simulink model "sm_excv_track1"  (R2026b)
settings: Solver=ode23t  StopTime=14  FixedStep=2e-4  AbsTol=1e-3
StartFcn:
  | tic
StopFcn:
  | Elapsed_Sim_Time = toc;
  | disp(['Elapsed Sim Time = ' num2str(Elapsed_Sim_Time)]);
undefined symbols (not defined in the file): Excv, X, Y, Z
libraries: sm_trackV_lib_terrain_contact x4, sm_lib x3, fl_lib x2, sm_excv_chassis_lib x2, nesl_utility x2, sm_trackV_lib_chain_underc_elem x1, sm_trackV_lib_chain_lower_frame_s46i1u2l7 x1, simulink x1
CloseFcn:
  | try,close(h1_sm_excv_track_single_terrain),end
  | clear h1_sm_excv_track_single_terrain
  | try,close(h2_sm_excv_track_single_terrain),end
  | clear h2_sm_excv_track_single_terrain
  | try,close(h3_sm_excv_track_single_terrain),end
  | clear h3_sm_excv_track_single_terrain
  | try,close(h4_sm_excv_track_single_terrain),end
  | clear h4_sm_excv_track_single_terrain
  | 
  | 
  | %clear simlog_sm_excv_track_single_road_plate
  | %clear logsout_sm_excv_track_single_road_plate
settings Model: Creator=evo  LastModifiedBy=smiller
settings SolverCC: AutoScaleAbsTol=off
settings DataIOCC: DSMLogging=off  ReturnWorkspaceOutputs=off  SaveOutput=off  SaveTime=off  SignalLoggingName=logsout_sm_excv_track1
settings DebuggingCC: SymbolicDimsDataTypeCodeGenerationDiagnostic=none
settings SFSimCC: CustomCodeUndefinedFunction=UseInterfaceOnly
settings RTWCC: DLArmComputeVersion=19.05
settings SimscapeCC: SimscapeLogLimitData=off  SimscapeLogName=simlog_sm_excv_track1  SimscapeLogSimulationStatistics=on  SimscapeLogType=all  SimscapeUseEnergyAccounting=off
settings DiagnosticsConfigSet: SimMechanicsConflictingReferenceFrames=none
settings ExplorerConfigSet: InternalSimMechanicsExplorerSettings="<ExplorerConfiguration><canonicalview>default</canonicalview><AnimationSetting><BasePlaybackSpeed>1.0</BasePlaybackSpeed><PlaybackSpeedFactor>0.25</PlaybackSpeedFactor></AnimationSetting><TilePanel><TileInfo><Tiles Columns=\"2\" Count=\"3\" Rows=\"2\"><Column Weight=\"0.5\"/><Column Weight=\"0.5\"/><Row Weight=\"0.5\"/><Row Weight=\"0.5\"/><Tile Height=\"1\" Width=\"2\" X=\"0\" Y=\"0\"/><Tile Height=\"1\" Width=\"1\" X=\"0\" Y=\"1\"/><Tile Height=\"1\" Width=\"1\" X=\"1\" Y=\"1\"/></Tiles></TileInfo><SceneInfo><SceneViewer><BGColor><R>1</R><G>1</G><B>1</B></BGColor><Camera><DoPerspective>on</DoPerspective><Position><X>4.57499999999987139</X><Y>-0.500000000001179279</Y><Z>0.554946553288407585</Z></Position><Center><X>4.15238173825940571</X><Y>0.406307787035579571</Y><Z>0.554946553288434119</Z></Center><Up><X>0</X><Y>0</Y><Z>1</Z></Up><ViewLimDist>1</ViewLimDist><YLim>0.466307658154998583</YLim><XLim>0.887968838401539839</XLim></Camera></SceneViewer><SceneViewer><BGColor><R>1</R><G>1</G><B>1</B></BGColor><Camera><DoPerspective>off</DoPerspective><Position><X>10.0004286080142499</X><Y>-63.1345143988139412</Y><Z>2.01677578846033079</Z></Position><Center><X>10.0000005340652702</X><Y>2.24533280857031059e-10</Y><Z>0.750000011139050793</Z></Center><Up><X>0.000675779963889239091</X><Y>0.0200606731361765434</Y><Z>0.999798536063523424</Z></Up><ViewLimDist>1</ViewLimDist><YLim>11.3757180156657967</YLim><XLim>10.6496083550913845</XLim></Camera></SceneViewer><SceneViewer><BGColor><R>1</R><G>1</G><B>1</B></BGColor><Camera><DoPerspective>on</DoPerspective><Position><X>1.68499999999974204</X><Y>-1.00000000000043432</Y><Z>0.55494655328839293</Z></Position><Center><X>1.68500000000000005</X><Y>-4.34319247233361239e-13</Y><Z>0.55494655328842224</Z></Center><Up><X>0</X><Y>0</Y><Z>1</Z></Up><ViewLimDist>1</ViewLimDist><YLim>0.466307658154998583</YLim><XLim>0.436543339549360365</XLim></Camera></SceneViewer></SceneInfo></TilePanel><MechEditorPanel><Cameras><Camera><Id>Camera1</Id><Value><Name>Track_CtrRear_AimFront</Name><NativeCamera><PositionTrackingFeature>Chassis.Camera_Frames.CamF_CtrRear_AimLF.R</PositionTrackingFeature><CenterTrackingFeature>Config.World_Frame.W</CenterTrackingFeature><UpVectorTrackingFeature>Config.World_Frame.W</UpVectorTrackingFeature><CenterTrackingOrigin>off</CenterTrackingOrigin><CenterTrackingDirection>+X</CenterTrackingDirection><UpVectorTrackingDirection>+Z</UpVectorTrackingDirection></NativeCamera></Value></Camera><Camera><Id>Camera2</Id><Value><Name>Track_Left_AimRight</Name><NativeCamera><PositionTrackingFeature>Chassis.Camera_Frames.CamF_Left_AimRight.R</PositionTrackingFeature><CenterTrackingFeature>Chassis.Camera_Frames.CamF_Left_AimRight.R</CenterTrackingFeature><UpVectorTrackingFeature>Config.World_Frame.W</UpVectorTrackingFeature><CenterTrackingOrigin>off</CenterTrackingOrigin><CenterTrackingDirection>+X</CenterTrackingDirection><UpVectorTrackingDirection>+Z</UpVectorTrackingDirection></NativeCamera></Value></Camera><Camera><Id>Camera3</Id><Value><Name>Track_Front_AimLR</Name><NativeCamera><PositionTrackingFeature>Chassis.Camera_Frames.CamF_Front_AimLR.R</PositionTrackingFeature><CenterTrackingFeature>Chassis.Camera_Frames.Transform_Aim_LR.F</CenterTrackingFeature><UpVectorTrackingFeature>Config.World_Frame.W</UpVectorTrackingFeature><CenterTrackingOrigin>off</CenterTrackingOrigin><CenterTrackingDirection>+X</CenterTrackingDirection><UpVectorTrackingDirection>+Z</UpVectorTrackingDirection></NativeCamera></Value></Camera><Camera><Id>Camera4</Id><Value><Name>Track_Right_AimLeftTL</Name><NativeCamera><PositionTrackingFeature>Chassis.Camera_Frames.CamF_Right_AimLeftTL.R</PositionTrackingFeature><CenterTrackingFeature>Chassis.Camera_Frames.CamF_Right_AimLeftTL.R</CenterTrackingFeature><UpVectorTrackingFeature>Config.World_Frame.W</UpVectorTrackingFeature><CenterTrackingOrigin>off</CenterTrackingOrigin><CenterTrackingDirection>+X</CenterTrackingDirection><UpVectorTrackingDirection>+Z</UpVectorTrackingDirection></NativeCamera></Value></Camera><Camera><Id>Camera5</Id><Value><Name>Track_Right_AimLeftTR</Name><NativeCamera><PositionTrackingFeature>Chassis.Camera_Frames.CamF_Right_AimLeftTR.R</PositionTrackingFeature><CenterTrackingFeature>Chassis.Camera_Frames.CamF_Right_AimLeftTR.R</CenterTrackingFeature><UpVectorTrackingFeature>Config.World_Frame.W</UpVectorTrackingFeature><CenterTrackingOrigin>off</CenterTrackingOrigin><CenterTrackingDirection>+X</CenterTrackingDirection><UpVectorTrackingDirection>+Z</UpVectorTrackingDirection></NativeCamera></Value></Camera><Camera><Id>Camera6</Id><Value><Name>Track_FR_AimFront</Name><NativeCamera><PositionTrackingFeature>Chassis.Camera_Frames.CamF_FR_Aim_Front_R</PositionTrackingFeature><CenterTrackingFeature>Chassis.Camera_Frames.CamF_FR_Aim_Front_R</CenterTrackingFeature><UpVectorTrackingFeature>Config.W</UpVectorTrackingFeature><CenterTrackingOrigin>off</CenterTrackingOrigin><CenterTrackingDirection>+X</CenterTrackingDirection><UpVectorTrackingDirection>+Z</UpVectorTrackingDirection></NativeCamera></Value></Camera></Cameras><GfxPanelCameraMap><MapElement CameraMLId=\"Camera6\" GfxPanelIndex=\"0\"/><MapElement CameraMLId=\"Camera4\" GfxPanelIndex=\"2\"/></GfxPanelCameraMap><VideoCreator><PlaybackSpeedRatio>1.0</PlaybackSpeedRatio><FrameRate>30</FrameRate><VideoFormat>Motion JPEG AVI</VideoFormat><FrameSize>auto</FrameSize></VideoCreator></MechEditorPanel></ExplorerConfiguration>"

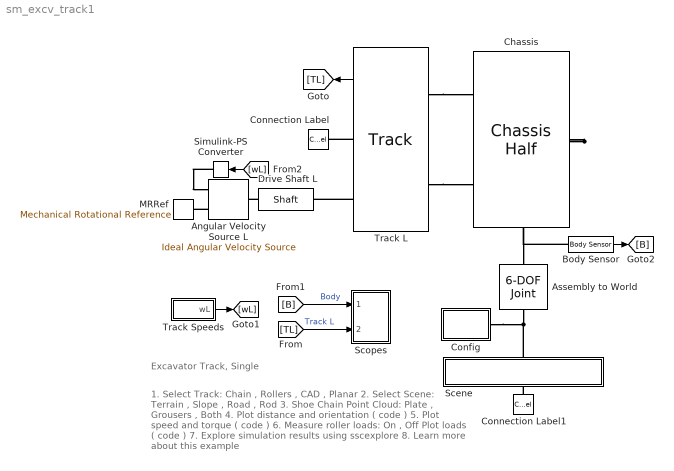
== system sm_excv_track1 ==
  note: Excavator Track, Single
  note: 1. Select Track: Chain , Rollers , CAD , Planar
      | 2. Select Scene: Terrain , Slope , Road , Rod
      | 3. Shoe Chain Point Cloud: Plate , Grousers , Both
      | 4. Plot distance and orientation ( code )
      | 5. Plot speed and torque ( code )
      | 6. Measure roller loads: On , Off Plot loads ( code )
      | 7. Explore simulation results using sscexplore
      | 8. Learn more about this example
  Angular Velocity Source L : fl_lib/Mechanical/Mechanical Sources/Ideal Angular Velocity Source
  Assembly to World : sm_lib/Joints/6-DOF Joint  JointMode=Normal  CompositeWrenchDir=FollowerOnBase  CompositeWrenchFrame=BaseFrame  SenseConstraintForce=off  SenseConstraintTorque=off  SenseTotalForce=off  SenseTotalTorque=off  PxPositionTargetSpecify=on  PxPositionTargetPriority=High  PxPositionTargetValue=0  PxPositionTargetValueUnits=m  PxVelocityTargetSpecify=off  PxVelocityTargetPriority=High  PxVelocityTargetValue=0  PxVelocityTargetValueUnits=m/s  PxEquilibriumPosition=0  PxEquilibriumPositionUnits=m  PxSpringStiffness=0  PxSpringStiffnessUnits=N/m  PxDampingCoefficient=0  PxDampingCoefficientUnits=N/(m/s)  PxLowerLimitSpecify=off  PxLowerLimitBound=-1  PxLowerLimitBoundUnits=m  PxLowerLimitStiffness=1e6  PxLowerLimitStiffnessUnits=N/m  PxLowerLimitDamping=1e3  PxLowerLimitDampingUnits=N/(m/s)  PxLowerLimitTransitionRegionWidth=1e-4  PxLowerLimitTransitionRegionWidthUnits=m  PxUpperLimitSpecify=off  PxUpperLimitBound=1  PxUpperLimitBoundUnits=m  PxUpperLimitStiffness=1e6  PxUpperLimitStiffnessUnits=N/m  PxUpperLimitDamping=1e3  PxUpperLimitDampingUnits=N/(m/s)  PxUpperLimitTransitionRegionWidth=1e-4  PxUpperLimitTransitionRegionWidthUnits=m  PxTorqueActuationMode=NoTorque  PxMotionActuationMode=ComputedMotion  PxSensePosition=off  PxSenseVelocity=off  PxSenseAcceleration=off  PxSenseTorqueForce=off  PxSenseLowerLimitTorqueForce=off  PxSenseUpperLimitTorqueForce=off  PyPositionTargetSpecify=on  PyPositionTargetPriority=High  PyPositionTargetValue=0  PyPositionTargetValueUnits=m  PyVelocityTargetSpecify=off  PyVelocityTargetPriority=High  PyVelocityTargetValue=0  PyVelocityTargetValueUnits=m/s  PyEquilibriumPosition=0  PyEquilibriumPositionUnits=m  PySpringStiffness=0  PySpringStiffnessUnits=N/m  PyDampingCoefficient=0  PyDampingCoefficientUnits=N/(m/s)  PyLowerLimitSpecify=off  PyLowerLimitBound=-1  PyLowerLimitBoundUnits=m  PyLowerLimitStiffness=1e6  PyLowerLimitStiffnessUnits=N/m  PyLowerLimitDamping=1e3  PyLowerLimitDampingUnits=N/(m/s)  PyLowerLimitTransitionRegionWidth=1e-4  PyLowerLimitTransitionRegionWidthUnits=m  PyUpperLimitSpecify=off  PyUpperLimitBound=1  PyUpperLimitBoundUnits=m  PyUpperLimitStiffness=1e6  PyUpperLimitStiffnessUnits=N/m  PyUpperLimitDamping=1e3  PyUpperLimitDampingUnits=N/(m/s)  PyUpperLimitTransitionRegionWidth=1e-4  PyUpperLimitTransitionRegionWidthUnits=m  PyTorqueActuationMode=NoTorque  PyMotionActuationMode=ComputedMotion  PySensePosition=off  PySenseVelocity=off  PySenseAcceleration=off  PySenseTorqueForce=off  PySenseLowerLimitTorqueForce=off  PySenseUpperLimitTorqueForce=off  PzPositionTargetSpecify=on  PzPositionTargetPriority=High  PzPositionTargetValue=Excv.Sprocket.sprocket_rPitch+0.2  PzPositionTargetValueUnits=m  PzVelocityTargetSpecify=off  PzVelocityTargetPriority=High  PzVelocityTargetValue=0  PzVelocityTargetValueUnits=m/s  PzEquilibriumPosition=0  PzEquilibriumPositionUnits=m  PzSpringStiffness=0  PzSpringStiffnessUnits=N/m  PzDampingCoefficient=0  PzDampingCoefficientUnits=N/(m/s)  PzLowerLimitSpecify=off  PzLowerLimitBound=-1  PzLowerLimitBoundUnits=m  PzLowerLimitStiffness=1e6  PzLowerLimitStiffnessUnits=N/m  PzLowerLimitDamping=1e3  PzLowerLimitDampingUnits=N/(m/s)  PzLowerLimitTransitionRegionWidth=1e-4  PzLowerLimitTransitionRegionWidthUnits=m  PzUpperLimitSpecify=off  PzUpperLimitBound=1  PzUpperLimitBoundUnits=m  PzUpperLimitStiffness=1e6  PzUpperLimitStiffnessUnits=N/m  PzUpperLimitDamping=1e3  PzUpperLimitDampingUnits=N/(m/s)  PzUpperLimitTransitionRegionWidth=1e-4  PzUpperLimitTransitionRegionWidthUnits=m  PzTorqueActuationMode=NoTorque  PzMotionActuationMode=ComputedMotion  PzSensePosition=off  PzSenseVelocity=off  PzSenseAcceleration=off  PzSenseTorqueForce=off  PzSenseLowerLimitTorqueForce=off  PzSenseUpperLimitTorqueForce=off  SphPositionTargetSpecify=off  SphPositionTargetPriority=High  SphPositionTargetRotationMethod=StandardAxis  SphPositionTargetFollAlignAxisA=+X  SphPositionTargetBaseAlignAxisA=+Y  SphPositionTargetFollAlignAxisB=+Y  SphPositionTargetBaseAlignAxisB=+Z  SphPositionTargetRotationStandardAxis=+Z  SphPositionTargetRotationAngle=180  SphPositionTargetRotationAngleUnits=deg  SphPositionTargetRotationArbitraryAxis=[0 0 1]  SphPositionTargetRotationSequenceAxes=FollowerAxes  SphPositionTargetRotationSequence=XYX  SphPositionTargetRotationSequenceAngles=[0 0 0]  SphPositionTargetRotationSequenceAnglesUnits=deg  SphPositionTargetRotationMatrix=[1 0 0; 0 1 0; 0 0 1]  SphPositionTargetQuaternion=[1 0 0 0]  SphVelocityTargetSpecify=off  SphVelocityTargetPriority=High  SphVelocityTargetValue=[0 0 0]  SphVelocityTargetValueUnits=deg/s  SphVelocityTargetInFollowerFrame=on  SphEqPosRotationMethod=None  SphEqPosFollAlignAxisA=+X  SphEqPosBaseAlignAxisA=+Y  SphEqPosFollAlignAxisB=+Y  SphEqPosBaseAlignAxisB=+Z  SphEqPosRotationStandardAxis=+Z  SphEqPosRotationAngle=0.0  SphEqPosRotationAngleUnits=deg  SphEqPosRotationArbitraryAxis=[0 0 1]  SphEqPosRotationSequenceAxes=FollowerAxes  SphEqPosRotationSequence=XYX  SphEqPosRotationSequenceAngles=[0 0 0]  SphEqPosRotationSequenceAnglesUnits=deg  SphEqPosRotationMatrix=[1 0 0; 0 1 0; 0 0 1]  SphEqPosQuaternion=[1 0 0 0]  SphSpringStiffness=0  SphSpringStiffnessUnits=N*m/deg  SphDampingCoefficient=0  SphDampingCoefficientUnits=N*m/(deg/s)  SphLowerLimitSpecify=off  SphLowerLimitBound=15  SphLowerLimitBoundUnits=deg  SphLowerLimitStiffness=1e4  SphLowerLimitStiffnessUnits=N*m/deg  SphLowerLimitDamping=10  SphLowerLimitDampingUnits=N*m/(deg/s)  SphLowerLimitTransitionRegionWidth=0.1  SphLowerLimitTransitionRegionWidthUnits=deg  SphUpperLimitSpecify=off  SphUpperLimitBound=45  SphUpperLimitBoundUnits=deg  SphUpperLimitStiffness=1e4  SphUpperLimitStiffnessUnits=N*m/deg  SphUpperLimitDamping=10  SphUpperLimitDampingUnits=N*m/(deg/s)  SphUpperLimitTransitionRegionWidth=0.1  SphUpperLimitTransitionRegionWidthUnits=deg  SphTorqueActuationMode=NoTorque  SphActuateTorqueX=off  SphActuateTorqueY=off  SphActuateTorqueZ=off  SphActuateTorque=off  SphActuationFrame=BaseFrame  SphSensePosition=off  SphSenseVelocityX=off  SphSenseVelocityY=off  SphSenseVelocityZ=off  SphSenseVelocity=off  SphSenseAccelerationX=off  SphSenseAccelerationY=off  SphSenseAccelerationZ=off  SphSenseAcceleration=off  SphSenseLowerLimitTorqueMag=off  SphSenseUpperLimitTorqueMag=off  SphSensingFrame=BaseFrame
  Body Sensor : sm_excv_chassis_lib/Body Sensor  offset_body_sensor=[0 0 0]
  Chassis : sm_excv_chassis_lib/Chassis Half  Camera=Excv.Chassis.Camera  offset_cg=Excv.Chassis.CGOffset  offset_axle=Excv.Chassis.AxleOffset  offset_sprk2axle_x=Excv.Frame.AxleX  offset_sprk2axle_y=Excv.Frame.AxleY  track_sep_ctr=Excv.Chassis.TrackSepCtr  chassis_mass=Excv.Chassis.Mass/2  chassis_moi=Excv.Chassis.MOI/2  chassis_poi=Excv.Chassis.POI/2
  Config : Subsystem
  Connection Label : ConnectionLabel  Label=GL
  Connection Label1 : ConnectionLabel  Label=GL
  Drive Shaft L : sm_trackV_lib_chain_underc_elem/Shaft  k_shaft=Excv.Drive.Shaft.k  b_shaft=Excv.Drive.Shaft.b
  MRRef : fl_lib/Mechanical/Rotational Elements/Mechanical Rotational Reference
  Scene : Subsystem  Variant=on  VariantControlMode=label  LabelModeActiveChoice=Terrain
      settings: AttributesFormatString=%<LabelModeActiveChoice>
      mask Display: disp(' ')
  Scopes : Subsystem
  Simulink-PS Converter : nesl_utility/Simulink-PS Converter  PhysicalDomain=network_engine_domain  SubClassName=ps_input  LeftPortType=input  RightPortType=output  PseudoPeriodic=off  Frequencies=[]  NoiseDistribution=none  NoiseParameters=[]  Unit=1  AffineConversion=off  FilteringAndDerivatives=provide  SimscapeFilterOrder=1  InputFilterTimeConstant=0.001  UdotUserProvided=0
  Track L : sm_trackV_lib_chain_lower_frame_s46i1u2l7/Track  LabelModeActiveChoice=ChainPts  popup_trackModel=Chain, Points  popup_leftOrRight=Left  popup_sense_roller=Actuator Torque
      settings: AttributesFormatString=|
      | %<popup_trackModel>
      | %<popup_sense_roller>
  Track Speeds : Subsystem  Variant=on  VariantControlMode=label  VariantControl=Fwd  LabelModeActiveChoice=Fwd
      settings: AttributesFormatString=%<LabelModeActiveChoice>
      mask Display: disp(' ')
  wires:
  [wL] -> Simulink-PS Converter/1
  Track L/1 -> [TL]
  [TL] -> Scopes/2(Track)  "Track L"
  [B] -> Scopes/1(Body)  "Body"
  Body Sensor/1 -> [B]
  Track Speeds/1(wL) -> [wL]
  connections:
  Assembly to World/LConn1 -- Scene/RConn1 -- Config/LConn1
  Chassis/RConn1 -- Body Sensor/LConn1 -- Assembly to World/RConn1
  Angular Velocity Source L/RConn2 -- MRRef/LConn1
  Drive Shaft L/LConn1 -- Angular Velocity Source L/LConn1
  Simulink-PS Converter/RConn1 -- Angular Velocity Source L/RConn1
  Track L/LConn2 -- Chassis/LConn2
  Track L/LConn1 -- Chassis/LConn1
  Track L/RConn2 -- Drive Shaft L/RConn1
  Track L/RConn1 -- Connection Label/LConn1
  Connection Label1/LConn1 -- Scene/LConn1

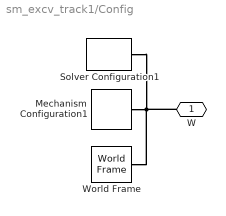
== system sm_excv_track1/Config ==
  Mechanism Configuration1 : sm_lib/Utilities/Mechanism Configuration  UniformGravity=Constant  GravityVector=[0 0 -9.80665]  GravityVectorUnits=m/s^2  LinearizationDelta=0.001  JointModeTransitionNonlinearIterations=2
  Solver Configuration1 : nesl_utility/Solver Configuration  PhysicalDomain=network_engine_domain  SubClassName=solver  LeftPortType=input  RightPortType=generic  Tones=[]  Harmonics=[]  SimulateNoise=off  Profile=off  UseLocalSampling=off  EnableSwitchedLinearOptims=on  FrequencyDomain=off  UseCCode=off  RelTol=0.001  AbsTol=0.001  MinStep=1e-09  ToWorkspace=off  RevertToSquareIcSolve=off  NumHomotopyIterations=100  PhasorMode=off  PhasorModeNumHarmonics=1  ConsistencySolver=NEWTON_FTOL  CanonicalOrdering=UNORDERED  OptimizeIntermediates=UNOPTIMIZED  MulticoreSolverChoice=BACKWARD_EULER  IndexReductionMethod=DerivativeReplacement  DoDC=off  ResidualTolerance=1e-09  ConsistencyTolSource=GLOBAL  ConsistencyAbsTol=0.001  ConsistencyRelTol=0.001  ConsistencyTolFactor=0.001  UseLocalSolver=off  LocalSolverChoice=NE_BACKWARD_EULER_ADVANCER  ResolveIndetEquations=on  FunctionEvalNumThread=1  LocalSolverSampleTime=0.001  DoFixedCost=off  MaxNonlinIter=3  MaxModeIter=2  ComputeImpulses=off  ImpulseIterations=2  LinearAlgebra=auto  LinearAlgebraNumThread=0  EquationFormulation=NE_TIME_EF  DelaysMemoryBudget=1024  AutomaticFiltering=on  FilteringTimeConstant=0.001  PartitionStorageMethod=AS_NEEDED  PartitionMemoryBudget=1024  PartitionMethod=BALANCED  MultibodyUseLocalSolver=off  MultibodyLocalSolverChoice=ODE1  MultibodyLocalSolverSampleTime=0.001
  World Frame : sm_lib/Frames and Transforms/World Frame
  W : PMIOPort  Side=Left
  connections:
  W/RConn1 -- Solver Configuration1/RConn1 -- Mechanism Configuration1/RConn1 -- World Frame/RConn1

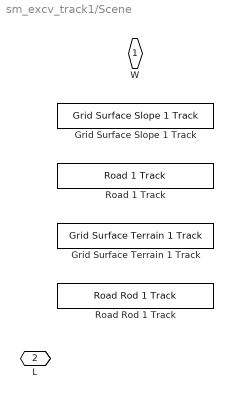
== system sm_excv_track1/Scene ==
  Grid Surface Slope 1 Track : sm_trackV_lib_terrain_contact/Grid Surface Slope 1 Track  VariantControl=Slope  road_len=Scene.Slope.road_len  road_wid=Scene.Slope.road_wid  slope_rise=Scene.Slope.slope_rise  slope_run=Scene.Slope.slope_run  slope_x0=Scene.Slope.slope_start  slope_xres=Scene.Slope.slope_xres  surface_clr=Scene.Slope.clr  surface_opc=Scene.Slope.opc  K_Road=Scene.Contact.Terrain.K  B_Road=Scene.Contact.Terrain.B  TW_Road=Scene.Contact.Terrain.TW  F_dyn_Road=Scene.Contact.Terrain.mud  F_stat_Road=Scene.Contact.Terrain.mus  CV_Road=Scene.Contact.Terrain.CV
  Grid Surface Terrain 1 Track : sm_trackV_lib_terrain_contact/Grid Surface Terrain 1 Track  SystemSampleTime=-1  VariantControl=Terrain  VariantActivationTime=update diagram  EmptyChoice=off  PassThrough=off  PassThroughVariantControl=(default)  EmptyChoiceVariantControl=(default)  AllowFlexibleInterface=on  Latency=0  AutoFrameSizeCalculation=off
  Road 1 Track : sm_trackV_lib_terrain_contact/Road 1 Track  SystemSampleTime=-1  VariantControl=Road  VariantActivationTime=update diagram  EmptyChoice=off  PassThrough=off  PassThroughVariantControl=(default)  EmptyChoiceVariantControl=(default)  AllowFlexibleInterface=on  Latency=0  AutoFrameSizeCalculation=off
  Road Rod 1 Track : sm_trackV_lib_terrain_contact/Road Rod 1 Track  SystemSampleTime=-1  VariantControl=Rod  VariantActivationTime=update diagram  EmptyChoice=off  PassThrough=off  PassThroughVariantControl=(default)  EmptyChoiceVariantControl=(default)  AllowFlexibleInterface=on  Latency=0  AutoFrameSizeCalculation=off
  W : PMIOPort  Side=Right
  L : PMIOPort  Port=2  Side=Left

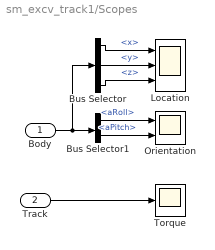
== system sm_excv_track1/Scopes ==
  Body : Inport
  Track : Inport  Port=2
  Bus Selector : BusSelector  OutputSignals=x,y,z
  Bus Selector1 : BusSelector  OutputSignals=aRoll,aPitch
  Location : Scope  NumInputPorts=3
      settings: ActiveDisplayYMinimum=-2.438  ActiveDisplayYMaximum=13.72233
  Orientation : Scope  NumInputPorts=2
      settings: ActiveDisplayYMinimum=-0.40552  ActiveDisplayYMaximum=0.36121  DataLoggingVariableName=ScopeData2
  Torque : Scope
  wires:
  Body/1 -> Bus Selector/1, Bus Selector1/1
  Bus Selector/3 -> Location/3  "<z>"
  Track/1 -> Torque/1
  Bus Selector1/1 -> Orientation/1  "<aRoll>"
  Bus Selector/2 -> Location/2  "<y>"
  Bus Selector/1 -> Location/1  "<x>"
  Bus Selector1/2 -> Orientation/2  "<aPitch>"

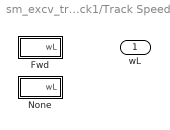
== system sm_excv_track1/Track Speeds ==
  Fwd : Subsystem  VariantControl=Fwd
  None : Subsystem  VariantControl=None
  wL : Outport

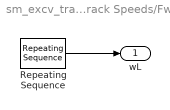
== system sm_excv_track1/Track Speeds/Fwd ==
  Repeating Sequence : simulink/Sources/Repeating Sequence  rep_seq_t=[0 2 2.01 40]  rep_seq_y=[0 0 3 3]
  wL : Outport
  wires:
  Repeating Sequence/1 -> wL/1

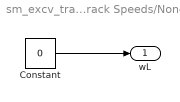
== system sm_excv_track1/Track Speeds/None ==
  Constant : Constant  Value=0
  wL : Outport
  wires:
  Constant/1 -> wL/1
